simulink model "Single_Phase_FCNPC_Rectifier"  (R2023b)
settings: Solver=ode45  StartTime=0.0  StopTime=0.5  RelTol=1e-3  EnableMultiTasking=on
libraries: spsSeriesRLCBranchLib x6, spsVoltageMeasurementLib x5, spsUniversalBridgeLib x4, simulink x2, spsACVoltageSourceLib x1, spsCurrentMeasurementLib x1, spsMeanLib x1, slpidlib x1, powerlib_extras x1, spsRMSLib x1, spsTHDLib x1, spspowerguiLib x1
settings Model: SimulationMode=accelerator  Creator=bzz  LastModifiedBy=Qu
settings SolverCC: ZeroCrossAlgorithm=Adaptive  AlgebraicLoopSolver=TrustRegion
settings DataIOCC: LimitDataPoints=on  ReturnWorkspaceOutputs=off
settings OptimizationCC: LifeSpan=inf
settings DebuggingCC: AlgebraicLoopMsg=none  IgnoredZcDiagnostic=none  UnconnectedInputMsg=warning  UnconnectedOutputMsg=warning  UnconnectedLineMsg=warning  AllowSymbolicDim=off  SFUnexpectedBacktrackingDiag=warning  SFNoUnconditionalDefaultTransitionDiag=warning  ArithmeticOperatorsInVariantConditions=warning
settings ModelReferenceCC: EnableRefExpFcnMdlSchedulingChecks=on  PropagateSignalLabelsOutOfModel=off
settings SFSimCC: SimUseLocalCustomCode=off  CustomCodeUndefinedFunction=UseInterfaceOnly
settings RTWCC: RTWUseLocalCustomCode=off  DLArmComputeVersion=19.05
settings CodeAppCC: StateflowObjectComments=on
settings GRTTargetCC: TargetLangStandard=C89/C90 (ANSI)
settings ConfigComp: CovMetricSettings=dw  CovSaveCumulativeToWorkspaceVar=on  CovSaveSingleToWorkspaceVar=on  CovExternalEMLEnable=off
settings SimscapeCC: SimscapeNormalizeSystem=off

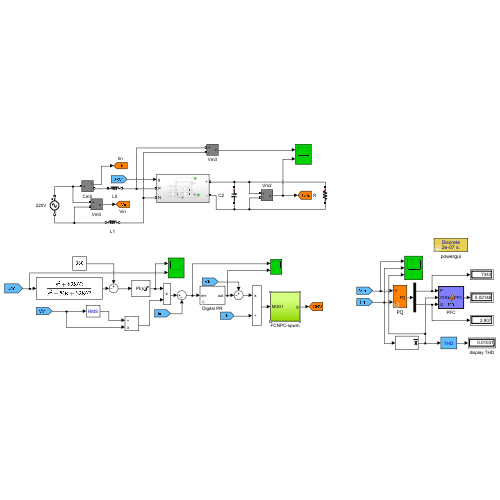
[thumbnail: Simulink's stored preview of the top-level diagram]
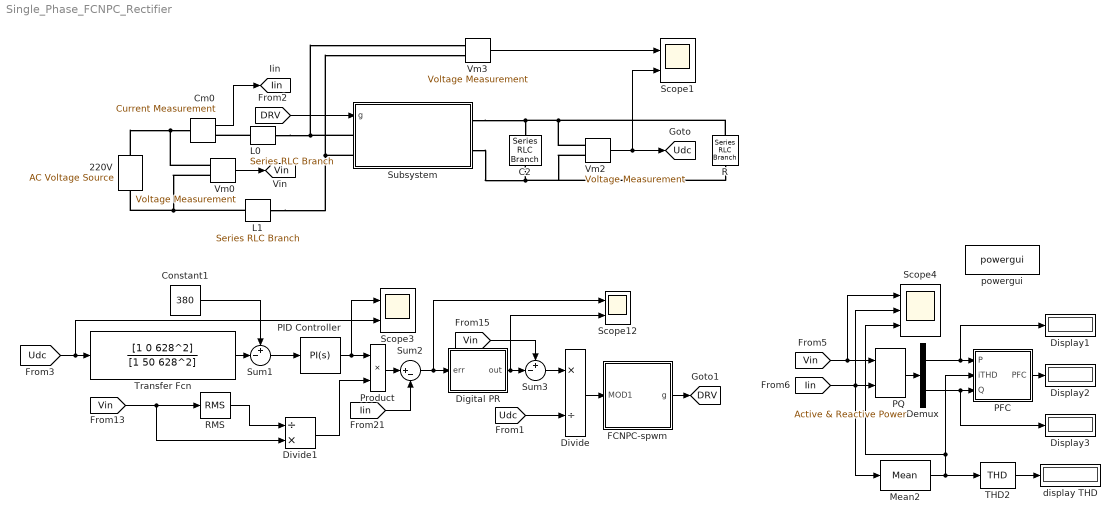
== system Single_Phase_FCNPC_Rectifier ==
  220V : spsACVoltageSourceLib/AC Voltage Source  Amplitude=225*1.4  Phase=0  Frequency=50  SampleTime=0  Measurements=None  BusType=swing  Pref=10e3  Qref=0  Qmin=-inf  Qmax=+inf
  C2 : spsSeriesRLCBranchLib/Series RLC Branch  LConnTagsString=__new0  RConnTagsString=__new0  BranchType=C  Resistance=0.1  Inductance=0  SetiL0=off  InitialCurrent=0  Capacitance=4e-3  Setx0=on  InitialVoltage=310  Measurements=None
  Cm0 : spsCurrentMeasurementLib/Current Measurement  PhasorSimulation=off  OutputType=Complex  PSBequivalent=0
  Constant1 : Constant  Value=380
  Demux : Demux  Outputs=2
  Digital PR : Subsystem  mask{Kp=8, Kr=100, Wc=5, Ts=1/40000, Upper=400, Lower=-400}
      mask DialogControl ParameterGroupVar Prompt: 参数
  Display1 : Display
  Display2 : Display
  Display3 : Display
  Divide : Product  Inputs=*/
  Divide1 : Product  Inputs=/*
  FCNPC-spwm : Subsystem
  L0 : spsSeriesRLCBranchLib/Series RLC Branch  LConnTagsString=__new0  RConnTagsString=__new0  BranchType=L  Resistance=0.05  Inductance=1e-4  SetiL0=off  InitialCurrent=0  Capacitance=inf  Setx0=off  InitialVoltage=0  Measurements=None
  L1 : spsSeriesRLCBranchLib/Series RLC Branch  LConnTagsString=__new0  RConnTagsString=__new0  BranchType=L  Resistance=0.05  Inductance=1e-4  SetiL0=off  InitialCurrent=0  Capacitance=inf  Setx0=off  InitialVoltage=0  Measurements=None
  Mean2 : spsMeanLib/Mean  Freq=20000  Vinit=0  Ts=0
  PFC : MATLAB Function  TreatAsAtomicUnit=on
  PID Controller : slpidlib/PID Controller  Controller=PI  Form=Parallel  TimeDomain=Continuous-time  UseExternalTs=off  SampleTime=-1  IntegratorMethod=Forward Euler  FilterMethod=Forward Euler  ControllerParametersSource=internal  P=0.5  I=30  UseKiTs=off  D=0.001  N=100  UseFilter=on  TunerSelectOption=Transfer Function Based (PID Tuner App)  InitialConditionSource=internal  InitialConditionForIntegrator=0  InitialConditionForFilter=0  DifferentiatorICPrevScaledInput=0  ExternalReset=none  TrackingMode=off  Kt=1  LimitOutput=on  SatLimitsSource=internal  UpperSaturationLimit=200  LowerSaturationLimit=-200  LinearizeAsGain=on  AntiWindupMode=clamping  Kb=1  LimitIntegrator=off  UpperIntegratorSaturationLimit=inf  LowerIntegratorSaturationLimit=-inf  POutMin=[]  POutMax=[]  IOutMin=[]  IOutMax=[]  DOutMin=[]  DOutMax=[]  NOutMin=[]  NOutMax=[]  SumOutMin=[]  SumOutMax=[]  SaturationOutMin=[]  SaturationOutMax=[]  PParamMin=[]  PParamMax=[]  IParamMin=[]  IParamMax=[]  DParamMin=[]  DParamMax=[]  NParamMin=[]  NParamMax=[]  KbParamMin=[]  KbParamMax=[]  KtParamMin=[]  KtParamMax=[]  KbOutMin=[]  KbOutMax=[]  KtOutMin=[]  KtOutMax=[]  IntegratorOutMin=[]  IntegratorOutMax=[]  FilterOutMin=[]  FilterOutMax=[]  SumI1OutMin=[]  SumI1OutMax=[]  SumI2OutMin=[]  SumI2OutMax=[]  SumI3OutMin=[]  SumI3OutMax=[]  SumI4OutMin=[]  SumI4OutMax=[]  SumDOutMin=[]  SumDOutMax=[]  DifferentiatorOutMin=[]  DifferentiatorOutMax=[]  FilterDiffOutCoefMin=[]  FilterDiffOutCoefMax=[]  ReciprocalOutMin=[]  ReciprocalOutMax=[]  SumDenOutMin=[]  SumDenOutMax=[]  SumNumOutMin=[]  SumNumOutMax=[]  DivideOutMin=[]  DivideOutMax=[]  UdiffTsProdOutMin=[]  UdiffTsProdOutMax=[]  NTsProdOutMin=[]  NTsProdOutMax=[]  UintegralTsProdOutMin=[]  UintegralTsProdOutMax=[]  UngainTsProdOutMin=[]  UngainTsProdOutMax=[]  ClampingZeroOutDataTypeStr=Inherit: Inherit via back propagation  ClampingZeroOutMin=[]  ClampingZeroOutMax=[]  FilterDenConstantOutDataTypeStr=Inherit: Inherit via back propagation  FilterDenConstantOutMin=[]  FilterDenConstantOutMax=[]  PCopyOutDataTypeStr=Inherit: Inherit via back propagation  PCopyOutMin=[]  PCopyOutMax=[]  NCopyOutDataTypeStr=Inherit: Inherit via back propagation  NCopyOutMin=[]  NCopyOutMax=[]  IntegratorContinuousStateAttributes=''  IntegratorStateMustResolveToSignalObject=off  IntegratorRTWStateStorageClass=Auto  FilterContinuousStateAttributes=''  FilterStateMustResolveToSignalObject=off  FilterRTWStateStorageClass=Auto  ParallelPVariant=InternalParameters  IdealPVariant=Disabled  IVariant=InternalParameters  DVariant=Disabled  IntegratorVariant=Continuous  SatVariant=Enabled  AWVariant=ContClampingParallel  PCopyVariant=Disabled  TRVariant=Disabled  FdbkBlocksVariant=Forward  IdealPFdbkVariant=Disabled  SatFdbkVariant=Disabled  DerivativeFilterVariant=Disabled  NVariant=Disabled  NCopyVariant=Disabled_SignalSpec  FilterICVariant=Disabled  IntegratorICVariant=InternalICs  ExternalResetVariant=Disabled  TRSumVariant=Passthrough  SumFdbkVariant=Disabled  SumVariant=Sum_PI  TsampFilterVariant=InternalTs  TsampNgainVariant=Passthrough  TsampIntegralVariant=Disabled_SignalSpec  ExternalSaturationOutDataTypeStr=Inherit: Same as second input
  PQ : powerlib_extras/Measurements/Active & Reactive Power  f1=50
  Product : Product
  R : spsSeriesRLCBranchLib/Series RLC Branch  LConnTagsString=__new0  RConnTagsString=__new0  BranchType=R  Resistance=20  Inductance=0  SetiL0=off  InitialCurrent=0  Capacitance=1e-5  Setx0=off  InitialVoltage=310  Measurements=None
  RMS : spsRMSLib/RMS  TrueRMS=on  Freq=50  RMSInit=220  Ts=0
  Scope1 : Scope  NumInputPorts=2
  Scope12 : Scope  NumInputPorts=2
  Scope3 : Scope  NumInputPorts=2
  Scope4 : Scope  NumInputPorts=3
  Subsystem : Subsystem
  Sum1 : Sum  Inputs=+-|
  Sum2 : Sum  Inputs=|+-
  Sum3 : Sum  Inputs=+-|
  THD2 : spsTHDLib/THD  Freq=50  Ts=0
  Transfer Fcn : TransferFcn  Numerator=[1 0 628^2]  Denominator=[1 50 628^2]
  Vm0 : spsVoltageMeasurementLib/Voltage Measurement  PhasorSimulation=off  OutputType=Complex  PSBequivalent=0
  Vm2 : spsVoltageMeasurementLib/Voltage Measurement  PhasorSimulation=off  OutputType=Complex  PSBequivalent=0
  Vm3 : spsVoltageMeasurementLib/Voltage Measurement  PhasorSimulation=off  OutputType=Complex  PSBequivalent=0
  display THD : Display
  powergui : spspowerguiLib/powergui  SimulationMode=Discrete  SampleTime=2e-7  frequency=60  Iterations=50  frequencyindice=0  Pbase=100e6  ErrMax=1e-4  UnitsV=kV  UnitsW=MW  buscounter=0  FunctionMessages=off  echomessages=off  EnableUseOfTLC=off  CurrentSourceSwitches=off  DisableSnubberDevices=off  DisableRonSwitches=off  DisableVfSwitches=off  DisplayEquations=off  AutomaticDiscreteSolvers=off  SolverType=Tustin/Backward Euler (TBE)  Interpol=off  ExternalGateDelay=off  methode=off  Ts=0  x0status=blocks  SPID=off  SwTol=0  HookPort=off  NonlinearTolerance=1e-4  nMaxIteration=100  ContinueOnMaxIteration=off  RestoreLinks=warning  ResistiveCurrentMeasurement=off  Frange=[0:2:500]  Ylog=off  Xlog=on  ShowGrid=off  save=off  variable=ZData  structure=QQQQQ  ZoomFFT=off  StartTime=0.5  cycles=15  DisplayStyle=1  fundamental=50  FreqAxis=off  MaxFrequency=1000  frequencyindicesteady=1  RmsSteady=1  display=off
  tag scope: DRV=global, Iin=global, Udc=global, Vin=global
  wires:
  Cm0/1 -> [Iin]
  Vm0/1 -> [Vin]
  PQ/1 -> Demux/1
  PFC/1(PFC) -> Display2/1
  Demux/1 -> Display1/1, PFC/1(P)
  Demux/2 -> Display3/1, PFC/3(Q)
  Sum1/1 -> PID Controller/1
  [Vin] -> Scope4/1, PQ/1
  [Iin] -> Mean2/1, Scope4/2, PQ/2
  [Vin] -> Divide1/2, RMS/1
  Mean2/1 -> THD2/1, PFC/2(iTHD), Scope4/3
  THD2/1 -> display THD/1
  Vm2/1 -> Scope1/2, [Udc]
  Digital PR/1(out) -> Sum3/2, Scope12/2
  [Iin] -> Sum2/2
  Sum3/1 -> Divide/1
  Sum2/1 -> Scope12/1, Digital PR/1(err)
  Product/1 -> Sum2/1
  [Udc] -> Divide/2
  PID Controller/1 -> Scope3/1, Product/1
  Divide1/1 -> Product/2
  FCNPC-spwm/1(g) -> [DRV]
  Vm3/1 -> Scope1/1
  [Udc] -> Transfer Fcn/1, Scope3/2
  Transfer Fcn/1 -> Sum1/2
  RMS/1 -> Divide1/1
  Constant1/1 -> Sum1/1
  [Vin] -> Sum3/1
  [DRV] -> Subsystem/1(g)
  Divide/1 -> FCNPC-spwm/1(MOD1)
  connections:
  Vm0/LConn1 -- Cm0/LConn1 -- 220V/RConn1
  L0/LConn1 -- Cm0/RConn1
  Vm2/LConn1 -- Subsystem/RConn1 -- C2/LConn1 -- R/LConn1
  Vm0/LConn2 -- L1/LConn1 -- 220V/LConn1
  L0/RConn1 -- Subsystem/LConn1 -- Vm3/LConn1
  Subsystem/LConn2 -- L1/RConn1 -- Vm3/LConn2
  Subsystem/RConn2 -- R/RConn1 -- Vm2/LConn2 -- C2/RConn1

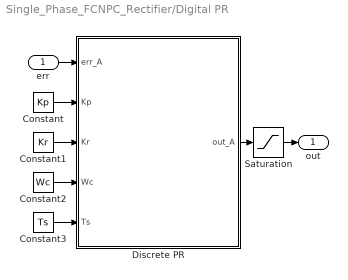
== system Single_Phase_FCNPC_Rectifier/Digital PR ==
  err : Inport
  Constant : Constant  Value=Kp
  Constant1 : Constant  Value=Kr
  Constant2 : Constant  Value=Wc
  Constant3 : Constant  Value=Ts
  Discrete PR : MATLAB Function  TreatAsAtomicUnit=on
  Saturation : Saturate  UpperLimit=Upper  LowerLimit=Lower
  out : Outport
  wires:
  Constant1/1 -> Discrete PR/3(Kr)
  Constant3/1 -> Discrete PR/5(Ts)
  Constant/1 -> Discrete PR/2(Kp)
  Constant2/1 -> Discrete PR/4(Wc)
  Discrete PR/1(out_A) -> Saturation/1
  Saturation/1 -> out/1
  err/1 -> Discrete PR/1(err_A)

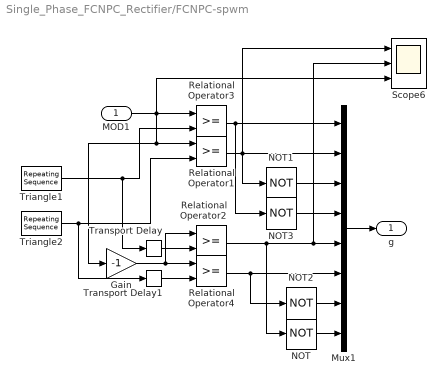
== system Single_Phase_FCNPC_Rectifier/FCNPC-spwm ==
  MOD1 : Inport
  Gain : Gain  Gain=-1
  Mux1 : Mux  Inputs=8
  NOT{,1..3} (4 alike) : Logic  Operator=NOT  IconShape=distinctive  AllPortsSameDT=off  OutDataTypeStr=boolean
  Relational Operator{1..4} (4 alike) : RelationalOperator  OutDataTypeStr=boolean  InputSameDT=off
  Scope6 : Scope  NumInputPorts=3
  Transport Delay : TransportDelay  DelayTime=1/20000/4
  Transport Delay1 : TransportDelay  DelayTime=1/20000/4
  Triangle1 : simulink/Sources/Repeating Sequence  rep_seq_t=[0 1/20000/2 1/20000]  rep_seq_y=[-1 1 -1]
  Triangle2 : simulink/Sources/Repeating Sequence  rep_seq_t=[0 1/20000/2 1/20000]  rep_seq_y=[1 -1 1]
  g : Outport
  wires:
  Mux1/1 -> g/1
  Relational Operator2/1 -> Mux1/5, Scope6/2, NOT/1
  NOT/1 -> Mux1/8
  NOT2/1 -> Mux1/7
  Gain/1 -> Relational Operator2/1, Relational Operator4/1
  Relational Operator4/1 -> Mux1/6, NOT2/1
  NOT1/1 -> Mux1/3
  NOT3/1 -> Mux1/4
  Relational Operator3/1 -> Mux1/1, NOT3/1
  Relational Operator1/1 -> Mux1/2, Scope6/1, NOT1/1
  Triangle2/1 -> Transport Delay1/1, Relational Operator1/2
  Triangle1/1 -> Relational Operator3/2, Transport Delay/1
  MOD1/1 -> Scope6/3, Relational Operator3/1, Relational Operator1/1, Gain/1
  Transport Delay/1 -> Relational Operator2/2
  Transport Delay1/1 -> Relational Operator4/2

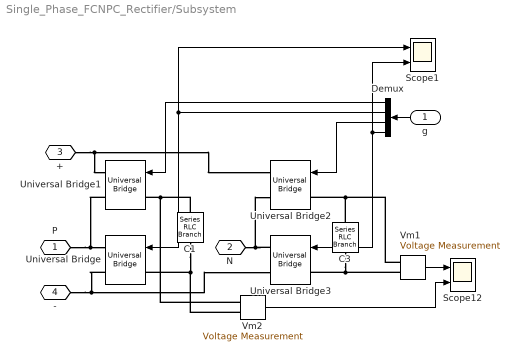
== system Single_Phase_FCNPC_Rectifier/Subsystem ==
  g : Inport
  C1 : spsSeriesRLCBranchLib/Series RLC Branch  LConnTagsString=__new0  RConnTagsString=__new0  BranchType=C  Resistance=0.1  Inductance=0  SetiL0=off  InitialCurrent=0  Capacitance=5e-5  Setx0=on  InitialVoltage=155  Measurements=None
  C3 : spsSeriesRLCBranchLib/Series RLC Branch  LConnTagsString=__new0  RConnTagsString=__new0  BranchType=C  Resistance=0.1  Inductance=0  SetiL0=off  InitialCurrent=0  Capacitance=5e-5  Setx0=on  InitialVoltage=155  Measurements=None
  Demux : Demux
  Scope1 : Scope  NumInputPorts=2
  Scope12 : Scope  NumInputPorts=2
  Universal Bridge{,1..3} (4 alike) : spsUniversalBridgeLib/Universal Bridge  Arms=1  SnubberResistance=1e6  SnubberCapacitance=inf  Device=IGBT / Diodes  Ron=1e-3  Lon=0  ForwardVoltages="[  1  1  ]"  ForwardVoltage=0  GTOparameters=[ 10e-6 , 20e-6 ]  IGBTparameters=[ 1e-6 , 2e-6 ]  Measurements=None  Measurements_2=None  converterType=Rectifier
  Vm1 : spsVoltageMeasurementLib/Voltage Measurement  PhasorSimulation=off  OutputType=Complex  PSBequivalent=0
  Vm2 : spsVoltageMeasurementLib/Voltage Measurement  PhasorSimulation=off  OutputType=Complex  PSBequivalent=0
  P : PMIOPort  Side=Left
  N : PMIOPort  Port=2  Side=Left
  + : PMIOPort  Port=3  Side=Right
  - : PMIOPort  Port=4  Side=Right
  wires:
  Demux/1 -> Universal Bridge1/1
  Demux/2 -> Universal Bridge/1, Scope1/1
  Demux/3 -> Universal Bridge2/1
  Demux/4 -> Universal Bridge3/1, Scope1/2
  Vm1/1 -> Scope12/1
  Vm2/1 -> Scope12/2
  g/1 -> Demux/1
  connections:
  C3/LConn1 -- Universal Bridge2/LConn1 -- Vm1/LConn1
  C3/RConn1 -- Universal Bridge3/LConn1 -- Vm1/LConn2
  Universal Bridge3/RConn1 -- N/RConn1 -- Universal Bridge2/RConn2
  Universal Bridge/RConn2 -- Universal Bridge3/RConn2 -- -/RConn1
  Universal Bridge1/RConn2 -- P/RConn1 -- Universal Bridge/RConn1
  C1/LConn1 -- Vm2/LConn1 -- Universal Bridge1/LConn1
  +/RConn1 -- Universal Bridge2/RConn1 -- Universal Bridge1/RConn1
  C1/RConn1 -- Vm2/LConn2 -- Universal Bridge/LConn1

== matlab function Single_Phase_FCNPC_Rectifier/PFC ==
  data: P input; iTHD input; PFC output; Q input
function PFC = fcn(P,iTHD,Q)
% This block supports an embeddable subset of the MATLAB language.
% See the help menu for details. 
PFC=(P/sqrt(P*P+Q*Q))/sqrt(1+iTHD*iTHD);

== matlab function Single_Phase_FCNPC_Rectifier/Digital PR/Discrete PR ==
  settings: updateMethod=DISCRETE  sampleTime=Ts
  data: err_A input; out_A output; Kp input; Kr input; Wc input; Ts input
function out_A  = fcn(err_A, Kp, Kr, Wc, Ts)

W0 = 50*2*pi;


persistent err_A1;
persistent err_A2;
persistent out_A1;
persistent out_A2;


%%对三相静态变量初始化
if isempty(err_A1)
    err_A1 = 0;
end
if isempty(err_A2)
    err_A2 = 0;
end
if isempty(out_A1)
    out_A1 = 0;
end
if isempty(out_A2)
    out_A2 = 0;
end


%%Discrete
t1 = Wc * Ts;
t2 = W0^2 * Ts^2;
t3 = t2 + 4*t1 + 4;

b0 = (Kp*t2 + 4*(Kp+Kr)*t1 + 4*Kp) / t3;
b1 = (2*Kp*t2 - 8*Kp) / t3;
b2 = (Kp*t2 + 4*Kp - 4*(Kp+Kr)*t1) / t3;
a1 = (2*t2 - 8) / t3;
a2 = (t2 - 4*t1 + 4) / t3;
%%限制输出
if b0>3000
    b0=0;
end
if b0<-3000
    b0=0;
end

%%计算输出量
out_A = b0*err_A + b1*err_A1 + b2*err_A2 - a1*out_A1 - a2*out_A2;
out_A2 = out_A1;
out_A1 = out_A;
err_A2 = err_A1;
err_A1 = err_A;
